simulink model "Tractor_HIT_Discrete"  (R2024a)
settings: Solver=ode1  StartTime=0.0  StopTime=60  FixedStep=0.001  RelTol=1e-3
values from neighbouring files (symbols this model uses):
  ANRtarget = 1.05    [Engine1204.sldd]    (also in Engine1204_init_r1.m; Engine2004.sldd; Engine2004_init.m; Engine3204.sldd)
  BackPrs = 3.0 4.2 5.5 7.0 8.5 10.0 11.5 12.5    [Engine1204.sldd]    (also in Engine1204_init_r1.m = [3.0, 4.2, 5.5, 7.0, 8.5, 10.0, 11.5, 12.5]; Engine2004.sldd = 3.0 4.2 5.5 7.0 8.5 10.0 11.5 12.5 13.5 14.5 15.0 15.5 16.0 ; Engine2004_init.m = [3.0,4.2,5.5,7.0,8.5,10.0,11.5,12.5,13.5,14.5,15.0,15.5,16.0; Engine3204.sldd = 3.0 4.5 6.0 7.5 9.0 10.5 12.0 13.0 13.8 14.4 14.8 15.2 15.6 )
  BackPrs_x = 50.0 100.0 150.0 200.0 250.0 300.0 350.0 400.0    [Engine1204.sldd]    (also in Engine1204_init_r1.m = [50:50:400]; Engine2004.sldd = 50.0 100.0 150.0 200.0 250.0 300.0 350.0 400.0 450.0 500.0 5; Engine2004_init.m = [50:50:800]; Engine3204.sldd = 100.0 200.0 300.0 400.0 500.0 600.0 700.0 800.0 900.0 1000.0)
  Bf = 0.38    [Engine1204.sldd]    (also in Engine2004.sldd; Engine3204.sldd)
  Br = 0.47    [Engine1204.sldd]    (also in Engine2004.sldd; Engine3204.sldd)
  BSFC = 320.0 285.0 275.0 280.0 290.0 300.0 310.0 260.0 225.0 215.0 220.0 228.0 240.0 250.0 235.0 208.0 202.0 205.0 212.0 222.0 232.0 230.0 205.0 200.0 204.0 210.0 220.0 230.0 232.0 207.0 203.0 206.0 213.0 224.0 235.0    [Engine1204.sldd]    (also in Engine1204_init_r1.m = [320,285,275,280,290,300,310; Engine2004.sldd = 315.0 280.0 270.0 275.0 285.0 295.0 305.0 255.0 220.0 210.0 ; Engine2004_init.m = [315,280,270,275,285,295,305; Engine3204.sldd = 310.0 275.0 265.0 270.0 280.0 290.0 300.0 250.0 215.0 205.0 )
  BSFC_x = 700.0 1200.0 1400.0 1600.0 1800.0 2000.0 2200.0    [Engine1204.sldd]    (also in Engine1204_init_r1.m = [700,1200,1400,1600,1800,2000,2200]; Engine2004.sldd = 800.0 1200.0 1400.0 1600.0 1800.0 2000.0 2200.0; Engine2004_init.m = [800,1200,1400,1600,1800,2000,2200]; Engine3204.sldd = 800.0 1000.0 1200.0 1400.0 1600.0 1800.0 2100.0)
  BSFC_y = 12.0 24.0 36.0 48.0 54.0    [Engine1204.sldd]    (also in Engine1204_init_r1.m = [12,24,36,48,54]; Engine2004.sldd = 20.0 40.0 60.0 80.0 100.0; Engine2004_init.m = [20,40,60,80,100]; Engine3204.sldd = 30.0 60.0 90.0 120.0 150.0)
  CO = 2.4 1.7 1.5 1.6 1.8 2.1 2.7 1.1 0.72 0.65 0.68 0.78 0.92 1.3 0.7 0.55 0.5 0.53 0.6 0.72 0.95 1.2 0.9 0.85 0.88 0.96 1.1 1.45 3.2 2.3 2.1 2.25 2.5 2.85 3.8    [Engine1204.sldd]    (also in Engine1204_init_r1.m = [; Engine2004.sldd = 2.3 1.63 1.44 1.54 1.73 2.02 2.56 1.05 0.68 0.61 0.64 0.74 0; Engine2004_init.m = [; Engine3204.sldd = 2.2 1.56 1.38 1.48 1.66 1.94 2.46 1.0 0.65 0.58 0.61 0.7 0.8)
  CO_x = 700.0 1200.0 1400.0 1600.0 1800.0 2000.0 2200.0    [Engine1204.sldd]    (also in Engine1204_init_r1.m = [700,1200,1400,1600,1800,2000,2200]; Engine2004.sldd = 800.0 1200.0 1400.0 1600.0 1800.0 2000.0 2200.0; Engine2004_init.m = [800,1200,1400,1600,1800,2000,2200]; Engine3204.sldd = 800.0 1000.0 1200.0 1400.0 1600.0 1800.0 2100.0)
  CO_y = 12.0 24.0 36.0 48.0 54.0    [Engine1204.sldd]    (also in Engine1204_init_r1.m = [12,24,36,48,54]; Engine2004.sldd = 20.0 40.0 60.0 80.0 100.0; Engine2004_init.m = [20,40,60,80,100]; Engine3204.sldd = 30.0 60.0 90.0 120.0 150.0)
  Df = 1.4    [Engine1204.sldd]    (also in Engine2004.sldd; Engine3204.sldd)
  dfmax = 0.1    [Engine1204.sldd]    (also in Engine2004.sldd; Engine3204.sldd)
  dfmin = 0.035    [Engine1204.sldd]    (also in Engine2004.sldd; Engine3204.sldd)
  DOCdPrs = 0.2 0.5 0.8 1.1 1.2    [Engine1204.sldd]    (also in Engine1204_init_r1.m = [0.2  0.5  0.8  1.1  1.2]; Engine2004.sldd = 0.25 0.55 0.85 1.15 1.3; Engine2004_init.m = [0.25,0.55,0.85,1.15,1.30]; Engine3204.sldd = 0.25 0.55 0.85 1.15 1.3 1.45)
  DOCdPrs_x = 50.0 150.0 250.0 350.0 400.0    [Engine1204.sldd]    (also in Engine1204_init_r1.m = [50  150  250  350  400]; Engine2004.sldd = 100.0 250.0 400.0 600.0 800.0; Engine2004_init.m = [100 250 400 600 800]; Engine3204.sldd = 100.0 250.0 400.0 600.0 800.0 1200.0)
  DPFdPrs = 0.3 0.5 0.7 0.9 0.6 1.0 1.4 1.8 0.9 1.5 2.1 2.6 1.2 2.0 2.7 2.8    [Engine1204.sldd]    (also in Engine1204_init_r1.m = [0.3  0.5  0.7  0.9; Engine2004.sldd = 0.35 0.6 0.85 1.1 0.7 1.15 1.6 2.0 1.05 1.7 2.3 2.5 1.4 2.2 ; Engine2004_init.m = [0.35,0.60,0.85,1.10; Engine3204.sldd = 0.35 0.7 1.05 1.4 1.7 2.0 2.2 2.4 2.55 2.65 2.7 2.75 0.6 1.1)
  DPFdPrs_x = 100.0 200.0 300.0 400.0    [Engine1204.sldd]    (also in Engine1204_init_r1.m = [100: 100 : 400]; Engine2004.sldd = 100.0 300.0 500.0 700.0; Engine2004_init.m = [100:200:700]; Engine3204.sldd = 100.0 200.0 300.0 400.0 500.0 600.0 700.0 800.0 900.0 1000.0)
  DPFdPrs_y = 0.0 6.0 12.0 20.0    [Engine1204.sldd]    (also in Engine1204_init_r1.m = [0 6 12 20 ]; Engine2004.sldd = 0.0 8.0 16.0 24.0; Engine2004_init.m = [0 8 16 24]; Engine3204.sldd = 0.0 10.0 20.0 30.0)
  DPFSootBurn = 0.0 0.0 0.0 0.0 0.0 0.2 0.4 0.6 0.8 1.0 1.2 2.4 3.6 4.8 6.0 6.0 12.0 18.0 24.0 30.0 12.0 24.0 36.0 48.0 60.0 20.0 40.0 60.0 80.0 100.0 22.0 44.0 66.0 88.0 110.0    [Engine1204.sldd]    (also in Engine1204_init_r1.m = [0,0,0,0,0; Engine2004.sldd = 0.0 0.0 0.0 0.0 0.0 0.5 1.0 1.5 2.0 2.5 3.0 6.0 9.0 12.0 15.; Engine2004_init.m = [0,0,0,0,0; Engine3204.sldd = 0.0 0.0 0.0 0.0 0.0 0.5 1.0 1.5 2.0 2.5 3.0 6.0 9.0 12.0 15.)
  DPFSootBurn_x = 100.0 200.0 300.0 400.0 500.0    [Engine1204.sldd]    (also in Engine1204_init_r1.m = [100,200,300,400,500]; Engine2004.sldd = 200.0 300.0 400.0 500.0 650.0; Engine2004_init.m = [200,300,400,500,650]; Engine3204.sldd = 200.0 300.0 400.0 500.0 650.0)
  DPFSootBurn_y = 400.0 450.0 500.0 550.0 600.0 650.0 680.0    [Engine1204.sldd]    (also in Engine1204_init_r1.m = [400,450,500,550,600,650,680]; Engine2004.sldd; Engine2004_init.m = [400,450,500,550,600,650,680]; Engine3204.sldd)
  Dr = 1.8    [Engine1204.sldd]    (also in Engine2004.sldd; Engine3204.sldd)
  drmax = 0.12    [Engine1204.sldd]    (also in Engine2004.sldd; Engine3204.sldd)
  drmin = 0.04    [Engine1204.sldd]    (also in Engine2004.sldd; Engine3204.sldd)
  EGRKi = 0.03    [Engine1204.sldd]    (also in Engine1204_init_r1.m; Engine2004.sldd; Engine2004_init.m; Engine3204.sldd)
  EGRKp = 3.5999999999999996    [Engine1204.sldd]    (also in Engine1204_init_r1.m = 3.6; Engine2004.sldd; Engine2004_init.m = 3.6; Engine3204.sldd)
  EGRMax = 1.0    [Engine1204.sldd]    (also in Engine1204_init_r1.m = 1; Engine2004.sldd; Engine2004_init.m = 1; Engine3204.sldd)
  EGRMin = 0.0    [Engine1204.sldd]    (also in Engine1204_init_r1.m = 0; Engine2004.sldd; Engine2004_init.m = 0; Engine3204.sldd)
  EGRRatio = 0.0 0.0 0.0 0.0 0.0 0.0 0.0 0.0 0.04 0.03 0.03 0.02 0.02 0.01 0.0 0.08 0.07 0.06 0.05 0.04 0.03 0.0 0.13 0.12 0.11 0.1 0.09 0.08 0.0 0.18 0.17 0.16 0.15 0.14 0.13 0.0 0.22 0.21 0.2 0.19 0.18 0.17    [Engine1204.sldd]    (also in Engine1204_init_r1.m = [; Engine2004.sldd; Engine2004_init.m = [; Engine3204.sldd)
  EGRRatio_x = 700.0 1200.0 1400.0 1600.0 1800.0 2000.0 2200.0    [Engine1204.sldd]    (also in Engine1204_init_r1.m = [700,1200,1400,1600,1800,2000,2200]; Engine2004.sldd = 800.0 1200.0 1400.0 1600.0 1800.0 2000.0 2200.0; Engine2004_init.m = [800,1200,1400,1600,1800,2000,2200]; Engine3204.sldd = 800.0 1000.0 1200.0 1400.0 1600.0 1800.0 2100.0)
  EGRRatio_y = 0.0 20.0 40.0 60.0 80.0 100.0    [Engine1204.sldd]    (also in Engine1204_init_r1.m = [0,20,40,60,80,100]; Engine2004.sldd; Engine2004_init.m = [0,20,40,60,80,100]; Engine3204.sldd)
  EGRTgt = 0.25 0.22 0.2 0.18 0.16 0.12 0.1 0.2 0.18 0.15 0.14 0.12 0.1 0.08 0.12 0.13 0.1 0.09 0.08 0.06 0.04 0.08 0.09 0.07 0.06 0.05 0.03 0.02 0.05 0.06 0.04 0.03 0.02 0.01 0.0    [Engine1204.sldd]    (also in Engine1204_init_r1.m = [0.25,0.22,0.20,0.18,0.16,0.12,0.10; Engine2004.sldd = 0.24 0.21 0.19 0.17 0.15 0.11 0.09 0.19 0.17 0.14 0.13 0.11 ; Engine2004_init.m = [0.24,0.21,0.19,0.17,0.15,0.11,0.09; Engine3204.sldd = 0.23 0.2 0.18 0.16 0.14 0.1 0.08 0.18 0.16 0.13 0.12 0.1 0.0)
  EGRTgt_x = 700.0 1200.0 1400.0 1600.0 1800.0 2000.0 2200.0    [Engine1204.sldd]    (also in Engine1204_init_r1.m = [700,1200,1400,1600,1800,2000,2200]; Engine2004.sldd = 800.0 1200.0 1400.0 1600.0 1800.0 2000.0 2200.0; Engine2004_init.m = [800,1200,1400,1600,1800,2000,2200]; Engine3204.sldd = 800.0 1000.0 1200.0 1400.0 1600.0 1800.0 2100.0)
  EGRTgt_y = 12.0 24.0 36.0 48.0 54.0    [Engine1204.sldd]    (also in Engine1204_init_r1.m = [12,24,36,48,54]; Engine2004.sldd = 20.0 40.0 60.0 80.0 100.0; Engine2004_init.m = [20,40,60,80,100]; Engine3204.sldd = 30.0 60.0 90.0 120.0 150.0)
  EGT = 197.0 257.0 287.0 297.0 287.0 267.0 247.0 267.0 357.0 397.0 407.0 392.0 367.0 347.0 337.0 437.0 472.0 482.0 462.0 437.0 407.0 367.0 477.0 502.0 512.0 492.0 467.0 437.0 377.0 487.0 510.0 520.0 500.0 477.0 447.0    [Engine1204.sldd]    (also in Engine1204_init_r1.m = [470,530,560,570,560,540,520; Engine2004.sldd = 187.0 247.0 277.0 287.0 277.0 257.0 237.0 257.0 347.0 387.0 ; Engine2004_init.m = [460,520,550,560,550,530,510; Engine3204.sldd = 307.0 327.0 338.0 327.0 307.0 277.0 237.0 322.0 337.0 332.0 )
  EGT_x = 700.0 1200.0 1400.0 1600.0 1800.0 2000.0 2200.0    [Engine1204.sldd]    (also in Engine1204_init_r1.m = [700,1200,1400,1600,1800,2000,2200]; Engine2004.sldd = 800.0 1200.0 1400.0 1600.0 1800.0 2000.0 2200.0; Engine2004_init.m = [800,1200,1400,1600,1800,2000,2200]; Engine3204.sldd = 800.0 1000.0 1200.0 1400.0 1600.0 1800.0 2100.0)
  EGT_y = 12.0 24.0 36.0 48.0 54.0    [Engine1204.sldd]    (also in Engine1204_init_r1.m = [12,24,36,48,54]; Engine2004.sldd = 20.0 40.0 60.0 80.0 100.0; Engine2004_init.m = [20,40,60,80,100]; Engine3204.sldd = 30.0 60.0 90.0 120.0 150.0)
  EngCsup = 0.35594 0.35501499999999997 0.353535 0.35242500000000004 0.351685 0.35150000000000003 0.35187 0.352795 0.35446 0.356865    [Engine1204.sldd]    (also in Engine2004.sldd; Engine3204.sldd)
  EngineSpdTgt = 700.0 850.0 1000.0 1150.0 1300.0 1450.0 1600.0 1750.0 1900.0 2050.0 2200.0    [Engine1204.sldd]    (also in Engine1204_init_r1.m = [700:150:2200]; Engine2004.sldd; Engine2004_init.m = [700:150:2200]; Engine3204.sldd = 800.0 930.0 1060.0 1190.0 1320.0 1450.0 1580.0 1710.0 1840.0)
  EngineSpdTgt_x = 0.0 10.0 20.0 30.0 40.0 50.0 60.0 70.0 80.0 90.0 100.0    [Engine1204.sldd]    (also in Engine1204_init_r1.m = [0:10:100]; Engine2004.sldd; Engine2004_init.m = [0:10:100]; Engine3204.sldd)
  EngineTrq = 70.0 110.0 130.0 125.0 115.0 100.0 85.0 180.0 280.0 320.0 310.0 285.0 250.0 220.0 260.0 370.0 410.0 395.0 365.0 320.0 280.0 300.0 420.0 450.0 435.0 400.0 350.0 300.0 310.0 435.0 460.0 445.0 410.0 355.0 305.0    [Engine1204.sldd]    (also in Engine1204_init_r1.m = [70,110,130,125,115,100,85; Engine2004.sldd = 130.0 200.0 240.0 230.0 210.0 180.0 150.0 320.0 480.0 550.0 ; Engine2004_init.m = [130,200,240,230,210,180,150; Engine3204.sldd = 210.0 320.0 380.0 360.0 330.0 290.0 240.0 510.0 760.0 870.0 )
  EngineTrq_x = 700.0 1200.0 1400.0 1600.0 1800.0 2000.0 2200.0    [Engine1204.sldd]    (also in Engine1204_init_r1.m = [700,1200,1400,1600,1800,2000,2200]; Engine2004.sldd = 800.0 1200.0 1400.0 1600.0 1800.0 2000.0 2200.0; Engine2004_init.m = [800,1200,1400,1600,1800,2000,2200]; Engine3204.sldd = 800.0 1000.0 1200.0 1400.0 1600.0 1800.0 2100.0)
  EngineTrq_y = 12.0 24.0 36.0 48.0 54.0    [Engine1204.sldd]    (also in Engine1204_init_r1.m = [12,24,36,48,54]; Engine2004.sldd = 20.0 40.0 60.0 80.0 100.0; Engine2004_init.m = [20,40,60,80,100]; Engine3204.sldd = 30.0 60.0 90.0 120.0 150.0)
  EngSpd = 800.0 1000.0 1200.0 1400.0 1600.0 1800.0 2000.0 2200.0 2400.0 2600.0    [Engine1204.sldd]    (also in Engine2004.sldd; Engine3204.sldd)
  EngTrq = 667.0 700.0 768.0 830.0 885.0 860.0 789.0 690.0 542.0 352.0    [Engine1204.sldd]    (also in Engine2004.sldd; Engine3204.sldd)
  etaCO = 0.0 0.0 0.0 0.0 0.6 0.45 0.3 0.15 0.92 0.85 0.75 0.6 0.98 0.95 0.9 0.82 0.99 0.97 0.94 0.88    [Engine1204.sldd]    (also in Engine1204_init_r1.m = [0.00	0.00	0.00	0.00; Engine2004.sldd; Engine2004_init.m = [0.00	0.00	0.00	0.00; Engine3204.sldd)
  etaCO_x = 10000.0 25000.0 40000.0 60000.0    [Engine1204.sldd]    (also in Engine1204_init_r1.m = [10000  25000  40000  60000]; Engine2004.sldd; Engine2004_init.m = [10000 25000 40000 60000]; Engine3204.sldd)
  etaCO_y = 120.0 200.0 280.0 360.0 450.0    [Engine1204.sldd]    (also in Engine1204_init_r1.m = [120, 200, 280, 360, 450]; Engine2004.sldd; Engine2004_init.m = [120,200,280,360,450]; Engine3204.sldd)
  etaHC = 0.0 0.0 0.0 0.0 0.5 0.35 0.2 0.1 0.88 0.8 0.68 0.5 0.96 0.92 0.86 0.75 0.98 0.95 0.91 0.83    [Engine1204.sldd]    (also in Engine1204_init_r1.m = [0.00	0.00	0.00	0.00; Engine2004.sldd; Engine2004_init.m = [0.00	0.00	0.00	0.00; Engine3204.sldd)
  etaHC_x = 10000.0 25000.0 40000.0 60000.0    [Engine1204.sldd]    (also in Engine1204_init_r1.m = [10000  25000  40000  60000]; Engine2004.sldd; Engine2004_init.m = [10000 25000 40000 60000]; Engine3204.sldd)
  etaHC_y = 120.0 200.0 280.0 360.0 450.0    [Engine1204.sldd]    (also in Engine1204_init_r1.m = [120, 200, 280, 360, 450]; Engine2004.sldd; Engine2004_init.m = [120,200,280,360,450]; Engine3204.sldd)
  etaNO2 = 0.0 0.0 0.0 0.0 0.2 0.15 0.1 0.05 0.4 0.33 0.25 0.18 0.55 0.48 0.4 0.3 0.6 0.53 0.45 0.35    [Engine1204.sldd]    (also in Engine1204_init_r1.m = [0.00	0.00	0.00	0.00; Engine2004.sldd; Engine2004_init.m = [0.00	0.00	0.00	0.00; Engine3204.sldd)
  etaNO2_x = 10000.0 25000.0 40000.0 60000.0    [Engine1204.sldd]    (also in Engine1204_init_r1.m = [10000  25000  40000  60000]; Engine2004.sldd; Engine2004_init.m = [10000 25000 40000 60000]; Engine3204.sldd)
  etaNO2_y = 120.0 200.0 280.0 360.0 450.0    [Engine1204.sldd]    (also in Engine1204_init_r1.m = [120, 200, 280, 360, 450]; Engine2004.sldd; Engine2004_init.m = [120,200,280,360,450]; Engine3204.sldd)
  etaPM = 0.995 0.992 0.988 0.98 0.996 0.994 0.99 0.985 0.997 0.995 0.992 0.988    [Engine1204.sldd]    (also in Engine1204_init_r1.m = [0.995  0.992  0.988  0.980; Engine2004.sldd; Engine2004_init.m = [0.995  0.992  0.988  0.980; Engine3204.sldd)
  etaPM_x = 10000.0 25000.0 40000.0 60000.0    [Engine1204.sldd]    (also in Engine1204_init_r1.m = [10000  25000  40000  60000]; Engine2004.sldd; Engine2004_init.m = [10000 25000 40000 60000]; Engine3204.sldd)
  etaPM_y = 150.0 300.0 450.0    [Engine1204.sldd]    (also in Engine1204_init_r1.m = [150, 300, 450]; Engine2004.sldd; Engine2004_init.m = [150,300,450]; Engine3204.sldd)
  FuelCyleMax = 40.0 45.0 50.0 52.0 54.0 50.0 60.0 65.0 66.0 68.0 52.0 64.0 66.0 67.0 68.0 50.0 62.0 64.0 65.0 66.0 48.0 58.0 60.0 61.0 62.0 42.0 50.0 52.0 53.0 54.0 38.0 44.0 46.0 47.0 48.0    [Engine1204.sldd]    (also in Engine1204_init_r1.m = [40,45,50,52,54; Engine2004.sldd = 65.0 75.0 82.0 88.0 92.0 75.0 88.0 94.0 98.0 102.0 78.0 92.0; Engine2004_init.m = [65,75,82,88,92; Engine3204.sldd = 95.0 110.0 125.0 140.0 155.0 110.0 130.0 145.0 160.0 175.0 1)
  FuelCyleMax_x = 80.0 140.0 200.0 260.0 320.0    [Engine1204.sldd]    (also in Engine1204_init_r1.m = [80,140,200,260,320]; Engine2004.sldd = 150.0 300.0 450.0 600.0 750.0; Engine2004_init.m = [150,300,450,600,750]; Engine3204.sldd = 250.0 500.0 750.0 1000.0 1300.0)
  FuelCyleMax_y = 700.0 1200.0 1400.0 1600.0 1800.0 2000.0 2200.0    [Engine1204.sldd]    (also in Engine1204_init_r1.m = [700,1200,1400,1600,1800,2000,2200]; Engine2004.sldd = 800.0 1200.0 1400.0 1600.0 1800.0 2000.0 2200.0; Engine2004_init.m = [800,1200,1400,1600,1800,2000,2200]; Engine3204.sldd = 800.0 1000.0 1200.0 1400.0 1600.0 1800.0 2100.0)
  FuelCyleMaxSw = 0.0    [Engine1204.sldd]    (also in Engine1204_init_r1.m = 0; Engine2004.sldd; Engine2004_init.m = 0; Engine3204.sldd)
  FuelCyleMin = 10.0    [Engine1204.sldd]    (also in Engine1204_init_r1.m = 10; Engine2004.sldd = 12.0; Engine2004_init.m = 12; Engine3204.sldd = 15.0)
  FuelKd = 0.0    [Engine1204.sldd]    (also in Engine1204_init_r1.m = 0; Engine2004.sldd; Engine2004_init.m = 0; Engine3204.sldd)
  FuelKi = 0.0162    [Engine1204.sldd]    (also in Engine1204_init_r1.m; Engine2004.sldd = 0.0198; Engine2004_init.m = 0.0198; Engine3204.sldd = 0.025199999999999997)
  FuelKp = 0.054    [Engine1204.sldd]    (also in Engine1204_init_r1.m; Engine2004.sldd = 0.066; Engine2004_init.m = 0.066; Engine3204.sldd = 0.083999999999999991)
  g = 9.81    [Engine1204.sldd]    (also in Engine2004.sldd; Engine3204.sldd)
  GearA = -2.9 0.0 6.0 2.5 1.0    [Engine1204.sldd]    (also in Engine2004.sldd; Engine3204.sldd)
  GearAC = -1.0 0.0 1.0 2.0 3.0    [Engine1204.sldd]    (also in Engine2004.sldd; Engine3204.sldd)
  GearFront = 17.574    [Engine1204.sldd]    (also in Engine2004.sldd; Engine3204.sldd)
  GearM = 2.33 1.75 1.4 1.0    [Engine1204.sldd]    (also in Engine2004.sldd; Engine3204.sldd)
  GearMC = 1.0 2.0 3.0 4.0    [Engine1204.sldd]    (also in Engine2004.sldd; Engine3204.sldd)
  GearRef = 14.6    [Engine1204.sldd]    (also in Engine2004.sldd; Engine3204.sldd)
  HC = 0.85 0.6 0.52 0.55 0.62 0.7 0.9 0.4 0.22 0.2 0.21 0.26 0.32 0.48 0.25 0.18 0.17 0.18 0.21 0.26 0.36 0.32 0.24 0.23 0.25 0.28 0.33 0.42 0.55 0.42 0.4 0.43 0.48 0.54 0.68    [Engine1204.sldd]    (also in Engine1204_init_r1.m = [; Engine2004.sldd = 0.82 0.58 0.5 0.53 0.6 0.68 0.87 0.38 0.21 0.19 0.2 0.24 0.3; Engine2004_init.m = [; Engine3204.sldd = 0.8 0.56 0.48 0.51 0.58 0.66 0.84 0.37 0.2 0.18 0.19 0.23 0.)
  HC_x = 700.0 1200.0 1400.0 1600.0 1800.0 2000.0 2200.0    [Engine1204.sldd]    (also in Engine1204_init_r1.m = [700,1200,1400,1600,1800,2000,2200]; Engine2004.sldd = 800.0 1200.0 1400.0 1600.0 1800.0 2000.0 2200.0; Engine2004_init.m = [800,1200,1400,1600,1800,2000,2200]; Engine3204.sldd = 800.0 1000.0 1200.0 1400.0 1600.0 1800.0 2100.0)
  HC_y = 12.0 24.0 36.0 48.0 54.0    [Engine1204.sldd]    (also in Engine1204_init_r1.m = [12,24,36,48,54]; Engine2004.sldd = 20.0 40.0 60.0 80.0 100.0; Engine2004_init.m = [20,40,60,80,100]; Engine3204.sldd = 30.0 60.0 90.0 120.0 150.0)
  hf = 0.35    [Engine1204.sldd]    (also in Engine2004.sldd; Engine3204.sldd)
  hr = 0.4    [Engine1204.sldd]    (also in Engine2004.sldd; Engine3204.sldd)
  IdleEngSpd = 700.0    [Engine1204.sldd]    (also in Engine2004.sldd; Engine3204.sldd)
  IdleThrottle = 0.3    [Engine1204.sldd]    (also in Engine2004.sldd; Engine3204.sldd)
  Inertia = 0.9    [Engine1204.sldd]    (also in Engine1204_init_r1.m; Engine2004.sldd = 1.4; Engine2004_init.m = 1.4; Engine3204.sldd = 2.0)
  Intake = 80.0 140.0 160.0 180.0 190.0 195.0 200.0 130.0 210.0 240.0 260.0 270.0 275.0 280.0 170.0 270.0 310.0 330.0 340.0 345.0 350.0 190.0 320.0 360.0 380.0 390.0 395.0 400.0 200.0 340.0 380.0 400.0 410.0 415.0 420.0    [Engine1204.sldd]    (also in Engine1204_init_r1.m = [80,140,160,180,190,195,200; Engine2004.sldd = 160.0 240.0 280.0 310.0 330.0 340.0 350.0 250.0 380.0 440.0 ; Engine2004_init.m = [160,240,280,310,330,340,350; Engine3204.sldd = 280.0 420.0 490.0 540.0 570.0 585.0 600.0 430.0 660.0 760.0 )
  Intake_x = 700.0 1200.0 1400.0 1600.0 1800.0 2000.0 2200.0    [Engine1204.sldd]    (also in Engine1204_init_r1.m = [700,1200,1400,1600,1800,2000,2200]; Engine2004.sldd = 800.0 1200.0 1400.0 1600.0 1800.0 2000.0 2200.0; Engine2004_init.m = [800,1200,1400,1600,1800,2000,2200]; Engine3204.sldd = 800.0 1000.0 1200.0 1400.0 1600.0 1800.0 2100.0)
  Intake_y = 12.0 24.0 36.0 48.0 54.0    [Engine1204.sldd]    (also in Engine1204_init_r1.m = [12,24,36,48,54]; Engine2004.sldd = 20.0 40.0 60.0 80.0 100.0; Engine2004_init.m = [20,40,60,80,100]; Engine3204.sldd = 30.0 60.0 90.0 120.0 150.0)
  IntakePrs = 1.0 1.1 1.22 1.35 1.48 1.6 1.7 1.0 1.12 1.24 1.37 1.5 1.62 1.72 1.0 1.13 1.25 1.38 1.51 1.63 1.73 1.0 1.14 1.26 1.39 1.52 1.64 1.74 1.0 1.15 1.27 1.4 1.53 1.65 1.75 1.0 1.16 1.28 1.41 1.54 1.66 1.76    [Engine1204.sldd]    (also in Engine1204_init_r1.m = [; Engine2004.sldd = 1.0 1.11 1.23 1.36 1.49 1.61 1.71 1.0 1.13 1.25 1.38 1.51 1.; Engine2004_init.m = [; Engine3204.sldd = 1.0 1.12 1.24 1.37 1.5 1.62 1.72 1.0 1.14 1.26 1.39 1.52 1.6)
  IntakePrs_x = 700.0 1200.0 1400.0 1600.0 1800.0 2000.0 2200.0    [Engine1204.sldd]    (also in Engine1204_init_r1.m = [700,1200,1400,1600,1800,2000,2200]; Engine2004.sldd = 800.0 1200.0 1400.0 1600.0 1800.0 2000.0 2200.0; Engine2004_init.m = [800,1200,1400,1600,1800,2000,2200]; Engine3204.sldd = 800.0 1000.0 1200.0 1400.0 1600.0 1800.0 2100.0)
  IntakePrs_y = 0.0 20.0 40.0 60.0 80.0 100.0    [Engine1204.sldd]    (also in Engine1204_init_r1.m = [0,20,40,60,80,100]; Engine2004.sldd; Engine2004_init.m = [0,20,40,60,80,100]; Engine3204.sldd)
  IntakePrsInit = 1.35    [Engine1204.sldd]    (also in Engine1204_init_r1.m; Engine2004.sldd; Engine2004_init.m; Engine3204.sldd)
  IntakeSw = 0    [Engine1204.sldd]    (also in Engine1204_init_r1.m = false; Engine2004.sldd; Engine2004_init.m = false; Engine3204.sldd)
  IntakeTC = 0.1    [Engine1204.sldd]    (also in Engine1204_init_r1.m; Engine2004.sldd; Engine2004_init.m; Engine3204.sldd)
  IntakeTemp = 25.0 28.0 30.0 32.0 34.0 36.0 38.0 25.0 38.0 40.0 42.0 44.0 46.0 48.0 25.0 48.0 50.0 52.0 54.0 56.0 58.0 25.0 58.0 60.0 62.0 64.0 66.0 68.0 25.0 66.0 68.0 70.0 72.0 74.0 76.0 25.0 72.0 74.0 76.0 78.0 80.0 82.0    [Engine1204.sldd]    (also in Engine1204_init_r1.m = [; Engine2004.sldd = 25.0 29.0 31.0 33.0 35.0 37.0 39.0 25.0 39.0 41.0 43.0 45.0 ; Engine2004_init.m = [; Engine3204.sldd = 25.0 30.0 32.0 34.0 36.0 38.0 40.0 25.0 40.0 42.0 44.0 46.0 )
  IntakeTemp_x = 700.0 1200.0 1400.0 1600.0 1800.0 2000.0 2200.0    [Engine1204.sldd]    (also in Engine1204_init_r1.m = [700,1200,1400,1600,1800,2000,2200]; Engine2004.sldd = 800.0 1200.0 1400.0 1600.0 1800.0 2000.0 2200.0; Engine2004_init.m = [800,1200,1400,1600,1800,2000,2200]; Engine3204.sldd = 800.0 1000.0 1200.0 1400.0 1600.0 1800.0 2100.0)
  IntakeTemp_y = 0.0 20.0 40.0 60.0 80.0 100.0    [Engine1204.sldd]    (also in Engine1204_init_r1.m = [0,20,40,60,80,100]; Engine2004.sldd; Engine2004_init.m = [0,20,40,60,80,100]; Engine3204.sldd)
  IntakeTempInit = 45.0    [Engine1204.sldd]    (also in Engine1204_init_r1.m = 45; Engine2004.sldd; Engine2004_init.m = 45; Engine3204.sldd)
  Jf = 180.0    [Engine1204.sldd]    (also in Engine2004.sldd; Engine3204.sldd)
  Jr = 450.0    [Engine1204.sldd]    (also in Engine2004.sldd; Engine3204.sldd)
  L = 2.75    [Engine1204.sldd]    (also in Engine2004.sldd; Engine3204.sldd)
  LiftTorque = 5000.0    [Engine1204.sldd]    (also in Engine2004.sldd; Engine3204.sldd)
  LoadTrqManu = 200.0    [Engine1204.sldd]    (also in Engine1204_init_r1.m = 200; Engine2004.sldd = 400.0; Engine2004_init.m = 400; Engine3204.sldd = 800.0)
  LoadTrqSW = 1    [Engine1204.sldd]    (also in Engine1204_init_r1.m = true; Engine2004.sldd; Engine2004_init.m = true; Engine3204.sldd = 0)
  M_I = 2500.0    [Engine1204.sldd]    (also in Engine2004.sldd; Engine3204.sldd)
  M_T = 6500.0    [Engine1204.sldd]    (also in Engine2004.sldd; Engine3204.sldd)
  MaxEngSpd = 2600.0    [Engine1204.sldd]    (also in Engine2004.sldd; Engine3204.sldd)
  NH3StoreMax = 0.0 1.2 2.0 2.4 2.2 1.7 1.1    [Engine1204.sldd]    (also in Engine1204_init_r1.m = [0  1.2  2.0  2.4  2.2  1.7  1.1]; Engine2004.sldd = 0.0 1.7 2.9 3.5 3.2 2.5 1.6; Engine2004_init.m = [0, 1.7, 2.9, 3.5, 3.2, 2.5, 1.6]; Engine3204.sldd = 0.0 2.2 3.8 4.5 4.2 3.3 2.1)
  NH3StoreMax_x = 180.0 220.0 260.0 300.0 340.0 380.0 420.0    [Engine1204.sldd]    (also in Engine1204_init_r1.m = [180  220  260  300  340  380  420]; Engine2004.sldd; Engine2004_init.m = [180 220 260 300 340 380 420]; Engine3204.sldd)
  NOx = 6.2 7.0 7.4 7.2 6.8 6.4 6.0 7.5 8.4 8.8 8.6 8.2 7.7 7.2 8.2 9.1 9.5 9.3 8.9 8.4 7.9 7.6 8.5 8.8 8.6 8.2 7.7 7.2 7.0 7.8 8.1 7.9 7.5 7.0 6.5    [Engine1204.sldd]    (also in Engine1204_init_r1.m = [6.2,7.0,7.4,7.2,6.8,6.4,6.0; Engine2004.sldd = 6.1 6.9 7.3 7.1 6.7 6.3 5.9 7.4 8.3 8.7 8.5 8.1 7.6 7.1 8.1 ; Engine2004_init.m = [6.1,6.9,7.3,7.1,6.7,6.3,5.9; Engine3204.sldd = 5.9 6.7 7.1 6.9 6.5 6.1 5.7 7.2 8.1 8.5 8.3 7.9 7.4 6.9 7.9 )
  NOx_x = 700.0 1200.0 1400.0 1600.0 1800.0 2000.0 2200.0    [Engine1204.sldd]    (also in Engine1204_init_r1.m = [700,1200,1400,1600,1800,2000,2200]; Engine2004.sldd = 800.0 1200.0 1400.0 1600.0 1800.0 2000.0 2200.0; Engine2004_init.m = [800,1200,1400,1600,1800,2000,2200]; Engine3204.sldd = 800.0 1000.0 1200.0 1400.0 1600.0 1800.0 2100.0)
  NOx_y = 12.0 24.0 36.0 48.0 54.0    [Engine1204.sldd]    (also in Engine1204_init_r1.m = [12,24,36,48,54]; Engine2004.sldd = 20.0 40.0 60.0 80.0 100.0; Engine2004_init.m = [20,40,60,80,100]; Engine3204.sldd = 30.0 60.0 90.0 120.0 150.0)
  NOxFac = 1.0 0.88 0.76 0.64 0.54 0.46 0.4    [Engine1204.sldd]    (also in Engine1204_init_r1.m = [1.00, 0.88, 0.76, 0.64, 0.54, 0.46, 0.40]; Engine2004.sldd; Engine2004_init.m = [1.00,0.88,0.76,0.64,0.54,0.46,0.40]; Engine3204.sldd)
  NOxFac_x = 0.0 0.05 0.1 0.15 0.19999999999999998 0.25 0.3    [Engine1204.sldd]    (also in Engine1204_init_r1.m = [0: 0.05 : 0.3]; Engine2004.sldd; Engine2004_init.m = [0:0.05:0.3]; Engine3204.sldd)
  NumCyl = 6.0    [Engine1204.sldd]    (also in Engine1204_init_r1.m = 6; Engine2004.sldd; Engine2004_init.m = 6; Engine3204.sldd)
  O2 = 16.5 16.0 15.8 15.5 15.2 14.8 14.5 13.0 12.2 11.8 11.5 11.2 10.8 10.5 9.5 8.6 8.0 7.7 7.4 7.0 6.7 7.0 6.2 5.6 5.3 5.0 4.7 4.4 6.0 5.3 4.8 4.5 4.2 4.0 3.8    [Engine1204.sldd]    (also in Engine1204_init_r1.m = [16.5,16.0,15.8,15.5,15.2,14.8,14.5; Engine2004.sldd = 16.3 15.8 15.6 15.3 15.0 14.6 14.3 12.8 12.0 11.6 11.3 11.0 ; Engine2004_init.m = [16.3,15.8,15.6,15.3,15.0,14.6,14.3; Engine3204.sldd = 16.0 15.5 15.3 15.0 14.7 14.3 14.0 12.5 11.7 11.3 11.0 10.7 )
  O2_x = 700.0 1200.0 1400.0 1600.0 1800.0 2000.0 2200.0    [Engine1204.sldd]    (also in Engine1204_init_r1.m = [700,1200,1400,1600,1800,2000,2200]; Engine2004.sldd = 800.0 1200.0 1400.0 1600.0 1800.0 2000.0 2200.0; Engine2004_init.m = [800,1200,1400,1600,1800,2000,2200]; Engine3204.sldd = 800.0 1000.0 1200.0 1400.0 1600.0 1800.0 2100.0)
  O2_y = 12.0 24.0 36.0 48.0 54.0    [Engine1204.sldd]    (also in Engine1204_init_r1.m = [12,24,36,48,54]; Engine2004.sldd = 20.0 40.0 60.0 80.0 100.0; Engine2004_init.m = [20,40,60,80,100]; Engine3204.sldd = 30.0 60.0 90.0 120.0 150.0)
  PM = 0.12 0.1 0.09 0.09 0.1 0.11 0.12 0.22 0.18 0.16 0.17 0.19 0.21 0.24 0.38 0.3 0.26 0.27 0.31 0.35 0.39 0.55 0.44 0.38 0.4 0.45 0.5 0.56 0.65 0.52 0.46 0.48 0.53 0.58 0.66    [Engine1204.sldd]    (also in Engine1204_init_r1.m = [0.12,0.10,0.09,0.09,0.10,0.11,0.12; Engine2004.sldd = 0.11 0.09 0.08 0.08 0.09 0.1 0.11 0.21 0.17 0.15 0.16 0.18 0; Engine2004_init.m = [0.11,0.09,0.08,0.08,0.09,0.10,0.11; Engine3204.sldd = 0.1 0.08 0.07 0.07 0.08 0.09 0.1 0.2 0.16 0.14 0.15 0.17 0.1)
  PM_x = 700.0 1200.0 1400.0 1600.0 1800.0 2000.0 2200.0    [Engine1204.sldd]    (also in Engine1204_init_r1.m = [700,1200,1400,1600,1800,2000,2200]; Engine2004.sldd = 800.0 1200.0 1400.0 1600.0 1800.0 2000.0 2200.0; Engine2004_init.m = [800,1200,1400,1600,1800,2000,2200]; Engine3204.sldd = 800.0 1000.0 1200.0 1400.0 1600.0 1800.0 2100.0)
  PM_y = 12.0 24.0 36.0 48.0 54.0    [Engine1204.sldd]    (also in Engine1204_init_r1.m = [12,24,36,48,54]; Engine2004.sldd = 20.0 40.0 60.0 80.0 100.0; Engine2004_init.m = [20,40,60,80,100]; Engine3204.sldd = 30.0 60.0 90.0 120.0 150.0)
  radps2rpm = 9.55    [Engine1204.sldd]    (also in Engine1204_init_r1.m; Engine2004.sldd; Engine2004_init.m; Engine3204.sldd)
  RailFuel = 400.0 600.0 700.0 700.0 650.0 600.0 550.0 600.0 800.0 900.0 900.0 850.0 800.0 750.0 700.0 1000.0 1100.0 1150.0 1100.0 1000.0 950.0 750.0 1200.0 1350.0 1350.0 1300.0 1200.0 1150.0 750.0 1300.0 1400.0 1450.0 1400.0 1300.0 1200.0    [Engine1204.sldd]    (also in Engine1204_init_r1.m = [400,600,700,700,650,600,550; Engine2004.sldd = 420.0 620.0 720.0 720.0 680.0 630.0 580.0 630.0 830.0 930.0 ; Engine2004_init.m = [420,620,720,720,680,630,580; Engine3204.sldd = 440.0 640.0 740.0 740.0 700.0 650.0 600.0 650.0 850.0 950.0 )
  RailFuel_x = 700.0 1200.0 1400.0 1600.0 1800.0 2000.0 2200.0    [Engine1204.sldd]    (also in Engine1204_init_r1.m = [700,1200,1400,1600,1800,2000,2200]; Engine2004.sldd = 800.0 1200.0 1400.0 1600.0 1800.0 2000.0 2200.0; Engine2004_init.m = [800,1200,1400,1600,1800,2000,2200]; Engine3204.sldd = 800.0 1000.0 1200.0 1400.0 1600.0 1800.0 2100.0)
  ... (+23 more)
undefined symbols (not defined in the file or in its folder): df, DiscIntNeverNeededParam, dr, MAP_AIR, MAP_EFF, MAP_EoCO, MAP_EoCO2, MAP_EoHC, MAP_EoNOx, MAP_EoPM, MAP_FUEL, MAP_FUELCMD, MAP_POWER, MAP_SPD, MAP_TEMPERATURE, NH3_MAX, R
libraries: simulink x9, slpidlib x5
(part 7 of 10)

== system Tractor_HIT_Discrete/WorkloadModel/Tires and Ground/CI_Calc ==
  Soil[-] : Inport
  moisture[%] : Inport  Port=2
  density[g/cm3] : Inport  Port=3
  Scene[-] : Inport  Port=4
  1 : Subsystem  Commented=on  TreatAsAtomicUnit=on
  2 : Subsystem  TreatAsAtomicUnit=on
  If : If  IfExpression=u1 == 0  ElseIfExpressions=u1 == 1,u1 == 2  ShowElse=off
  If Action Subsystem : Subsystem  TreatAsAtomicUnit=on
  If Action Subsystem1 : Subsystem  TreatAsAtomicUnit=on
  Merge : Merge  Inputs=3
  CI[kPa] : Outport
  wires:
  Soil[-]/1 -> If/1
  moisture[%]/1 -> [moisture]
  density[g/cm3]/1 -> [density]
  [moisture] -> If Action Subsystem/1(moisture[%])
  [density] -> If Action Subsystem/2(density[g/cm3])
  Merge/1 -> CI[kPa]/1
  If/1 -> If Action Subsystem/Action
  If Action Subsystem/1(CI) -> Merge/1
  If Action Subsystem1/1(CI) -> Merge/2
  [moisture] -> If Action Subsystem1/1(moisture[%])
  [density] -> If Action Subsystem1/2(density[g/cm3])
  2/1(CI) -> Merge/3
  [moisture] -> 2/1(moisture[%])
  [density] -> 2/2(density[g/cm3])
  If/3 -> 2/Action
  If/2 -> If Action Subsystem1/Action
  Scene[-]/1 -> If Action Subsystem/3(Scene[-])

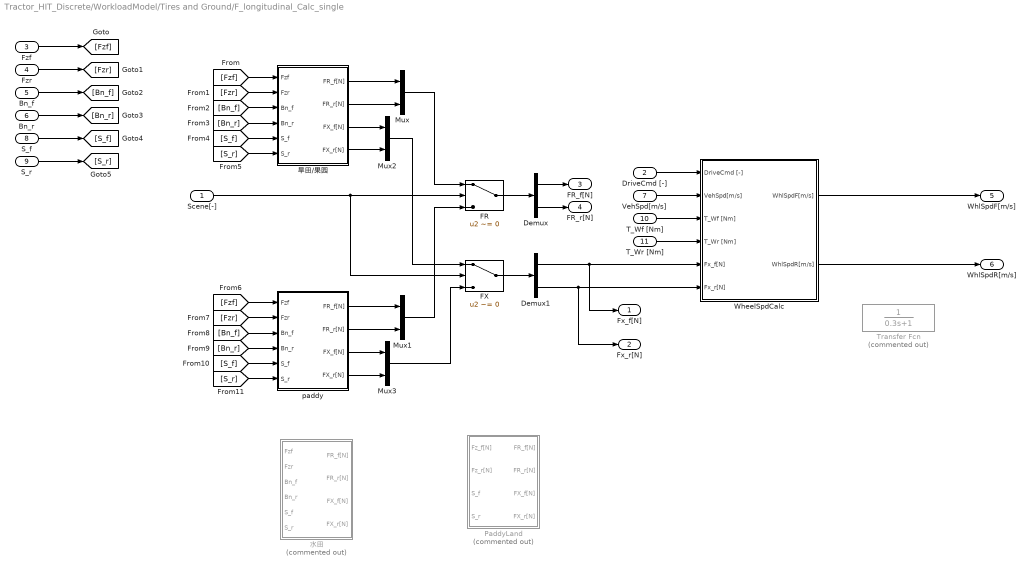
== system Tractor_HIT_Discrete/WorkloadModel/Tires and Ground/F_longitudinal_Calc_single ==
  Scene[-] : Inport
  DriveCmd [-] : Inport  Port=2
  Fzf : Inport  Port=3
  Fzr : Inport  Port=4
  Bn_f : Inport  Port=5
  Bn_r : Inport  Port=6
  VehSpd[m/s] : Inport  Port=7
  S_f : Inport  Port=8
  S_r : Inport  Port=9
  T_Wf [Nm] : Inport  Port=10
  T_Wr [Nm] : Inport  Port=11
  Demux : Demux  Outputs=2
  Demux1 : Demux  Outputs=2
  FR : Switch  Criteria=u2 ~= 0  SaturateOnIntegerOverflow=off  InputSameDT=off
  FX : Switch  Criteria=u2 ~= 0  SaturateOnIntegerOverflow=off  InputSameDT=off
  Mux{,1..3} (4 alike) : Mux  Inputs=2
  PaddyLand : Subsystem  Commented=on
  Transfer Fcn : TransferFcn  Commented=on  Denominator=[0.3 1]
  WheelSpdCalc : Subsystem
  paddy : Subsystem
  旱田/果园 : Subsystem
  水田 : Subsystem  Commented=on
  Fx_f[N] : Outport
  Fx_r[N] : Outport  Port=2
  FR_f[N] : Outport  Port=3
  FR_r[N] : Outport  Port=4
  WhlSpdF[m/s] : Outport  Port=5
  WhlSpdR[m/s] : Outport  Port=6
  wires:
  DriveCmd [-]/1 -> WheelSpdCalc/1(DriveCmd [-])
  T_Wf [Nm]/1 -> WheelSpdCalc/3(T_Wf [Nm])
  VehSpd[m/s]/1 -> WheelSpdCalc/2(VehSpd[m/s])
  T_Wr [Nm]/1 -> WheelSpdCalc/4(T_Wr [Nm])
  Scene[-]/1 -> FR/2, FX/2
  FR/1 -> Demux/1
  旱田/果园/1(FR_f[N]) -> Mux/1
  旱田/果园/2(FR_r[N]) -> Mux/2
  paddy/1(FR_f[N]) -> Mux1/1
  paddy/2(FR_r[N]) -> Mux1/2
  Mux1/1 -> FR/3
  Mux/1 -> FR/1
  Demux/1 -> FR_f[N]/1
  Demux/2 -> FR_r[N]/1
  FX/1 -> Demux1/1
  Demux1/1 -> Fx_f[N]/1, WheelSpdCalc/5(Fx_f[N])
  Demux1/2 -> Fx_r[N]/1, WheelSpdCalc/6(Fx_r[N])
  旱田/果园/3(FX_f[N]) -> Mux2/1
  旱田/果园/4(FX_r[N]) -> Mux2/2
  paddy/3(FX_f[N]) -> Mux3/1
  paddy/4(FX_r[N]) -> Mux3/2
  Mux3/1 -> FX/3
  Mux2/1 -> FX/1
  Fzf/1 -> [Fzf]
  Fzr/1 -> [Fzr]
  S_r/1 -> [S_r]
  S_f/1 -> [S_f]
  Bn_r/1 -> [Bn_r]
  Bn_f/1 -> [Bn_f]
  [Bn_r] -> 旱田/果园/4(Bn_r)
  [S_f] -> 旱田/果园/5(S_f)
  [S_r] -> 旱田/果园/6(S_r)
  [Bn_f] -> 旱田/果园/3(Bn_f)
  [Fzr] -> 旱田/果园/2(Fzr)
  [Fzf] -> 旱田/果园/1(Fzf)
  [Fzf] -> paddy/1(Fzf)
  [Fzr] -> paddy/2(Fzr)
  [Bn_f] -> paddy/3(Bn_f)
  [S_r] -> paddy/6(S_r)
  [S_f] -> paddy/5(S_f)
  [Bn_r] -> paddy/4(Bn_r)
  WheelSpdCalc/1(WhlSpdF[m/s]) -> WhlSpdF[m/s]/1
  WheelSpdCalc/2(WhlSpdR[m/s]) -> WhlSpdR[m/s]/1

== system Tractor_HIT_Discrete/WorkloadModel/Tires and Ground/Fz_Calc_single ==
  pitch_angle[rad] : Inport
  Add : Sum
  Add1 : Sum
  Constant : Constant  Value=M_T
  Constant1 : Constant  Value=g
  Constant2 : Constant  Value=L
  Constant3 : Constant  Value=L
  Constant4 : Constant  Value=Xof
  Constant5 : Constant  Value=Xor
  Constant6 : Constant  Value=Rr
  Constant7 : Constant  Value=Zor
  Cos : Trigonometry  Operator=cos
  Display : Display
  Display1 : Display
  Divide : Product  Inputs=*/
  Divide1 : Product  Inputs=*/
  Fz_Calc : Subsystem  Commented=on
  Gain : Gain  Gain=0.5
  Gain1 : Gain  Gain=0.5
  Product : Product
  Product2 : Product  Inputs=3
  Product3 : Product  Inputs=3
  Product4 : Product  Inputs=3
  Sin : Trigonometry
  Subtract : Sum  Inputs=+-
  Fzf : Outport
  Fzr : Outport  Port=2
  wires:
  pitch_angle[rad]/1 -> Sin/1, Cos/1
  Constant/1 -> Product/1
  Constant1/1 -> Product/2
  Constant2/1 -> Divide/2
  Constant3/1 -> Divide1/2
  Constant5/1 -> Product2/1
  Cos/1 -> Product2/2, Product3/2
  Product3/1 -> Subtract/1
  Product2/1 -> Add/1
  Constant4/1 -> Product3/3
  Add/1 -> Divide1/1
  Subtract/1 -> Divide/1
  Sin/1 -> Product4/3
  Product4/1 -> Add/2, Subtract/2
  Constant6/1 -> Add1/1
  Constant7/1 -> Add1/2
  Add1/1 -> Product4/2
  Divide1/1 -> Display1/1, Gain/1
  Divide/1 -> Display/1, Gain1/1
  Gain/1 -> Fzf/1
  Gain1/1 -> Fzr/1
  Product/1 -> Product4/1, Product3/1, Product2/3

== system Tractor_HIT_Discrete/WorkloadModel/Tires and Ground/Slip_calc ==
  VehSpd [m/s] : Inport
  WhlSpdF[m/s] : Inport  Port=2
  WhlSpdR[m/s] : Inport  Port=3
  Add : Sum
  Add1 : Sum
  Add2 : Sum  Inputs=+-
  Add3 : Sum  Inputs=+-
  Constant : Constant  Value=eps
  Divide : Product  Inputs=*/
  Divide1 : Product  Inputs=*/
  Max : MinMax  Function=max  Inputs=2
  Max1 : MinMax  Function=max  Inputs=2
  Scope : Scope  NumInputPorts=3
  SlipF [-] : Outport
  SlipR [-] : Outport  Port=2
  wires:
  Add3/1 -> Divide1/1
  Max/1 -> Add1/1
  Add2/1 -> Divide/1
  Constant/1 -> Add/2, Add1/2
  Max1/1 -> Add/1
  Add/1 -> Divide1/2
  Add1/1 -> Divide/2
  WhlSpdF[m/s]/1 -> Scope/2, Max/2, Add2/1
  VehSpd [m/s]/1 -> Scope/1, Max/1, Max1/1, Add3/2, Add2/2
  WhlSpdR[m/s]/1 -> Max1/2, Scope/3, Add3/1
  Divide1/1 -> SlipR [-]/1
  Divide/1 -> SlipF [-]/1

== system Tractor_HIT_Discrete/WorkloadModel/Tires and Ground/SlopeResistance_Calc ==
  note: SlopeResis_Calc
  Terrain[-] : Inport
  Constant2 : Constant  Value=M_T
  Fcn : Fcn  Expr=sin(u)
  Gain6 : Gain  Gain=pi/180
  Gain8 : Gain  Gain=g
  Multiport Switch : MultiPortSwitch  DataPortOrder=Zero-based contiguous  zeroidx=on  SaturateOnIntegerOverflow=off  InputSameDT=off
  Product2 : Product
  Sine Wave : Sin  Amplitude=5  Frequency=20  SampleTime=0
  Sine Wave1 : Sin  Amplitude=15  Frequency=10  SampleTime=0
  Sine Wave2 : Sin  Amplitude=30  Frequency=5  SampleTime=0
  SlopeResis[N] : Outport
  pitch_angle[rad] : Outport  Port=2
  wires:
  Sine Wave2/1 -> Multiport Switch/4
  Fcn/1 -> Product2/2
  Gain6/1 -> pitch_angle[rad]/1, Fcn/1
  Gain8/1 -> Product2/1
  Constant2/1 -> Gain8/1
  Multiport Switch/1 -> Gain6/1
  Sine Wave/1 -> Multiport Switch/2
  Sine Wave1/1 -> Multiport Switch/3
  Product2/1 -> SlopeResis[N]/1
  Terrain[-]/1 -> Multiport Switch/1

== system Tractor_HIT_Discrete/WorkloadModel/Transmission/EngSpdCalc ==
  Gear_R[-] : Inport
  DriveWhlSpd[m/s] : Inport  Port=2
  DriveWhlR[m] : Inport  Port=3
  Constant1 : Constant  Value=9.55
  Divide : Product  Inputs=*/
  Product : Product  Inputs=3
  Saturation1 : Saturate  UpperLimit=MaxEngSpd  LowerLimit=IdleEngSpd
  Scope2 : Scope  NumInputPorts=4
  EngSpd [rpm] : Outport
  wires:
  Product/1 -> Scope2/2, Divide/1
  Constant1/1 -> Product/3
  DriveWhlR[m]/1 -> Divide/2
  Divide/1 -> Scope2/3, Saturation1/1
  DriveWhlSpd[m/s]/1 -> Scope2/1, Product/2
  Gear_R[-]/1 -> Product/1
  Saturation1/1 -> Scope2/4, EngSpd [rpm]/1

== system Tractor_HIT_Discrete/WorkloadModel/Transmission/GearBox ==
  GearCmd[-] : Inport
  EngTrq [Nm] : Inport  Port=2
  1-D Lookup Table1 : Lookup_n-D  NumberOfTableDimensions=1  BreakpointsForDimension1=GearMC  Table=GearM  InternalRulePriority=Speed  RndMeth=Simplest
  1-D Lookup Table2 : Lookup_n-D  NumberOfTableDimensions=1  BreakpointsForDimension1=GearAC  Table=GearA  InternalRulePriority=Speed  RndMeth=Simplest
  1-D Lookup Table3 : Lookup_n-D  NumberOfTableDimensions=1  BreakpointsForDimension1=SlowFastC  Table=SlowFastGear  InternalRulePriority=Speed  RndMeth=Simplest
  Bus Selector : BusSelector  OutputSignals=FastSlowCmd,GearMCmd,GearACmd
  Effi : Constant  Value=TransEff
  Product1 : Product  Inputs=3
  Product2 : Product  Inputs=3
  Scope1 : Scope  NumInputPorts=3
  GearTrq [Nm] : Outport
  Gear [-] : Outport  Port=2
  wires:
  EngTrq [Nm]/1 -> Scope1/2, Product2/1
  Product1/1 -> Product2/2, Scope1/1, Gear [-]/1
  Product2/1 -> Scope1/3, GearTrq [Nm]/1
  Bus Selector/3 -> 1-D Lookup Table2/1  "<GearACmd>"
  GearCmd[-]/1 -> Bus Selector/1
  Bus Selector/1 -> 1-D Lookup Table3/1  "<FastSlowCmd>"
  Bus Selector/2 -> 1-D Lookup Table1/1  "<GearMCmd>"
  Effi/1 -> Product2/3
  1-D Lookup Table3/1 -> Product1/1
  1-D Lookup Table1/1 -> Product1/2
  1-D Lookup Table2/1 -> Product1/3

== system Tractor_HIT_Discrete/WorkloadModel/Transmission/GearBox2Axle ==
  note: 主减速比
  note: 前桥减速比
  DriveCmd [-] : Inport
  GearTrq [Nm] : Inport  Port=2
  Gear [-] : Inport  Port=3
  PTOTrq [Nm] : Inport  Port=4
  LiftTrq [Nm] : Inport  Port=5
  4WD : Subsystem  TreatAsAtomicUnit=on
  Constant : Constant  Value=GearFront
  Constant1 : Constant  Value=GearRef
  Constant2 : Constant  Value=GearFront
  Constant3 : Constant  Value=GearRef
  If : If  IfExpression=u1 == 0  ElseIfExpressions=u1 == 1  ShowElse=off
  Merge : Merge
  Merge1 : Merge
  Product{,1..3} (4 alike) : Product
  RWD : Subsystem  TreatAsAtomicUnit=on
  Scope1 : Scope  NumInputPorts=3
  Scope2 : Scope  NumInputPorts=4
  Subtract : Sum  Inputs=+--
  AxlTrqF [Nm] : Outport
  AxlTrqR [Nm] : Outport  Port=2
  Gear_F[-] : Outport  Port=3
  Gear_R[-] : Outport  Port=4
  wires:
  RWD/2(AxlTrqR [Nm]) -> Merge/1
  4WD/1(AxlTrqF [Nm]) -> Merge1/2
  DriveCmd [-]/1 -> If/1
  If/2 -> 4WD/Action
  PTOTrq [Nm]/1 -> Subtract/2
  RWD/1(AxlTrqF [Nm]) -> Merge1/1
  If/1 -> RWD/Action
  GearTrq [Nm]/1 -> Scope2/1, Subtract/1
  4WD/2(AxlTrqR [Nm]) -> Merge/2
  LiftTrq [Nm]/1 -> Subtract/3
  Subtract/1 -> Scope2/2, RWD/1(AxlTrq [Nm]), 4WD/1(AxlTrq [Nm])
  Gear [-]/1 -> Scope1/1, Product/1, Product1/1
  Product1/1 -> Scope1/2, Gear_F[-]/1
  Product/1 -> Scope1/3, Gear_R[-]/1
  Constant/1 -> Product1/2
  Constant1/1 -> Product/2
  Merge1/1 -> Product2/1
  Product2/1 -> Scope2/3, AxlTrqF [Nm]/1
  Constant2/1 -> Product2/2
  Constant3/1 -> Product3/2
  Merge/1 -> Product3/1
  Product3/1 -> Scope2/4, AxlTrqR [Nm]/1

== system Tractor_HIT_Discrete/WorkloadModel/Transmission/Motion ==
  EngineTrq_Nm : Inport
  LoadTrq_Nm : Inport  Port=2
  Add : Sum  Inputs=+-
  Constant : Constant  Value=Inertia
  Constant1 : Constant  Value=radps2rpm
  Divide : Product  Inputs=*/
  Integrator : Integrator  InitialCondition=SpeedInit  LimitOutput=on  UpperSaturationLimit=2400  LowerSaturationLimit=700
  Mux : Mux  Inputs=2
  Product : Product
  Scope2 : Scope  NumInputPorts=2
  EngineSpd_rpm : Outport
  wires:
  EngineTrq_Nm/1 -> Mux/1, Add/1
  LoadTrq_Nm/1 -> Mux/2, Add/2
  Add/1 -> Divide/1
  Constant/1 -> Divide/2
  Constant1/1 -> Product/2
  Product/1 -> Integrator/1
  Divide/1 -> Product/1
  Integrator/1 -> Scope2/2, EngineSpd_rpm/1
  Mux/1 -> Scope2/1

== system Tractor_HIT_Discrete/Engine/Engine/AftertreatmentModel/DOC ==
  note: GHSV = 气体空速，Gas Hourly Space Velocity
  ExhMassFlow_kg/h : Inport
  EGT_c : Inport  Port=2
  ExhPrs_kpa : Inport  Port=3
  O2_pct : Inport  Port=4
  NOx_kg/h : Inport  Port=5
  HC_kg/h : Inport  Port=6
  CO_kg/h : Inport  Port=7
  PM_kg/h : Inport  Port=8
  Add{,1..2,4} (4 alike) : Sum  Inputs=+-
  Add3 : Sum  Inputs=+++
  Constant : Constant
  Constant1 : Constant
  Constant2 : Constant
  DOCdPrs : Lookup_n-D  NumberOfTableDimensions=1  BreakpointsForDimension1=DOCdPrs_x  Table=DOCdPrs  ExtrapMethod=Clip  InternalRulePriority=Speed  RndMeth=Simplest
  GHSV : Subsystem
  Gain : Gain  Gain=20
  Gain1 : Gain  Gain=25
  Product{,1..3} (4 alike) : Product
  Scope : Scope  NumInputPorts=4
  Terminator : Terminator
  eta_CO : Lookup_n-D  BreakpointsForDimension1=etaCO_x  BreakpointsForDimension2=etaCO_y  Table=etaCO  ExtrapMethod=Clip  InternalRulePriority=Speed  RndMeth=Simplest
      settings: InputPortMap=u0,u1
  eta_HC : Lookup_n-D  BreakpointsForDimension1=etaHC_x  BreakpointsForDimension2=etaHC_y  Table=etaHC  ExtrapMethod=Clip  InternalRulePriority=Speed  RndMeth=Simplest
      settings: InputPortMap=u0,u1
  eta_NO2 : Lookup_n-D  BreakpointsForDimension1=etaNO2_x  BreakpointsForDimension2=etaNO2_y  Table=etaNO2  ExtrapMethod=Clip  InternalRulePriority=Speed  RndMeth=Simplest
      settings: InputPortMap=u0,u1
  DOC_Flow_kg/h : Outport
  DOC_Temp_c : Outport  Port=2
  DOC_NO2Frac : Outport  Port=3
  DOC_PM_kg/h : Outport  Port=4
  DOC_NO2_kg/h : Outport  Port=5
  DOC_NO_kg/h : Outport  Port=6
  DOC_Prs_kpa : Outport  Port=7
  DOC_dPrs_kpa : Outport  Port=8
  DOC_HC_kg/h : Outport  Port=9
  DOC_CO_kg/h : Outport  Port=10
  wires:
  PM_kg/h/1 -> DOC_PM_kg/h/1
  ExhPrs_kpa/1 -> DOCdPrs/1, Add4/1, GHSV/3(ExhPrs_kpa)
  EGT_c/1 -> Add3/3, eta_NO2/2, eta_HC/2, eta_CO/2, GHSV/2(EGT_c)
  ExhMassFlow_kg/h/1 -> GHSV/1(ExhMassFlow_kg/h), DOC_Flow_kg/h/1
  GHSV/1(GHSV_1/h) -> eta_NO2/1, eta_HC/1, eta_CO/1
  eta_CO/1 -> Gain/1, Add/2
  Constant/1 -> Add/1
  Add/1 -> Product/2
  CO_kg/h/1 -> Product/1
  Product/1 -> Scope/1, DOC_CO_kg/h/1  "DOC_CO_kg"
  Product1/1 -> Scope/2, DOC_HC_kg/h/1  "DOC_HC_kg/h"
  Add1/1 -> Product1/2
  Constant1/1 -> Add1/1
  eta_HC/1 -> Gain1/1, Add1/2
  HC_kg/h/1 -> Product1/1
  NOx_kg/h/1 -> Product3/1, Product2/2
  Product2/1 -> Scope/3, DOC_NO2_kg/h/1  "DOC_NO2_kg/h"
  Product3/1 -> Scope/4, DOC_NO_kg/h/1  "DOC_NO_kg/h"
  eta_NO2/1 -> DOC_NO2Frac/1, Product2/1, Add2/2
  Constant2/1 -> Add2/1
  Add2/1 -> Product3/2
  O2_pct/1 -> Terminator/1
  DOCdPrs/1 -> Add4/2, DOC_dPrs_kpa/1
  Gain/1 -> Add3/1
  Gain1/1 -> Add3/2
  Add3/1 -> DOC_Temp_c/1
  Add4/1 -> DOC_Prs_kpa/1

== system Tractor_HIT_Discrete/Engine/Engine/AftertreatmentModel/DPF ==
  DOC_Flow_kg/h : Inport
  DOC_Temp_c : Inport  Port=2
  DOC_NO2Frac : Inport  Port=3
  DOC_PM_kg/h : Inport  Port=4
  DOC_NO2_kg/h : Inport  Port=5
  DOC_NO_kg/h : Inport  Port=6
  DOC_Prs_kpa : Inport  Port=7
  DPF_regen_req : Inport  Port=8
  Add : Sum  Inputs=+-
  Add1 : Sum
  Add4 : Sum  Inputs=-+
  Constant : Constant
  DPFdPrs : Lookup_n-D  BreakpointsForDimension1=DPFdPrs_x  BreakpointsForDimension2=DPFdPrs_y  Table=DPFdPrs  InternalRulePriority=Speed  RndMeth=Simplest
      settings: InputPortMap=u0,u1
  GHSV : Subsystem
  Product : Product
  Scope : Scope  NumInputPorts=2
  SootLoad : Subsystem
  eta_PM : Lookup_n-D  BreakpointsForDimension1=etaPM_x  BreakpointsForDimension2=etaPM_y  Table=etaPM  InternalRulePriority=Speed  RndMeth=Simplest
      settings: InputPortMap=u0,u1
  DPF_Flow_kg/h : Outport
  DPF_Temp_c : Outport  Port=2
  DPF_Prs_kpa : Outport  Port=3
  DPF_NOx_kg/h : Outport  Port=4
  DPF_NO2Frac : Outport  Port=5
  DPF_PM_kg/h : Outport  Port=6
  DPF_SootLoad_g : Outport  Port=7
  DPF_dPrs_kpa : Outport  Port=8
  wires:
  DOC_NO2Frac/1 -> DPF_NO2Frac/1
  DOC_Flow_kg/h/1 -> DPFdPrs/1, DPF_Flow_kg/h/1, GHSV/1(ExhMassFlow_kg/h), SootLoad/2(DOC_Flow_kg/h)
  DOC_Temp_c/1 -> GHSV/2(EGT_c), SootLoad/3(DOC_Temp_c), DPF_Temp_c/1, eta_PM/2
  DOC_Prs_kpa/1 -> Add4/2, GHSV/3(ExhPrs_kpa)
  GHSV/1(GHSV_1/h) -> eta_PM/1
  Product/1 -> Scope/1, DPF_PM_kg/h/1
  Constant/1 -> Add/1
  eta_PM/1 -> SootLoad/4(eta_PM), Add/2
  Add/1 -> Product/1
  DOC_PM_kg/h/1 -> Scope/2, SootLoad/5(DOC_PM_kg/h), Product/2
  DPF_regen_req/1 -> SootLoad/1(DPF_regen_req)
  SootLoad/1(SootLoad_g) -> DPFdPrs/2, DPF_SootLoad_g/1
  DPFdPrs/1 -> Add4/1, DPF_dPrs_kpa/1
  Add4/1 -> DPF_Prs_kpa/1
  DOC_NO2_kg/h/1 -> Add1/1
  DOC_NO_kg/h/1 -> Add1/2
  Add1/1 -> DPF_NOx_kg/h/1

== system Tractor_HIT_Discrete/Engine/Engine/AftertreatmentModel/SCR ==
  note: 0.0001~0.001 kg/h 这个量级
  note: SCR 载体内部积存的氨，是积分状态；
  note: 氨逃逸
  note: 实际尿素喷射流量
  note: 尿素喷射执行
  DPF_Flow_kg/h : Inport
  DPF_Temp_c : Inport  Port=2
  DPF_Prs_kpa : Inport  Port=3
  DPF_NOx_kg/h : Inport  Port=4
  mUREA_target : Inport  Port=5
  Add1 : Sum  Inputs=+--
  Add2 : Sum  Inputs=+-
  Add3 : Sum  Inputs=+-
  Integrator : Integrator  UpperSaturationLimit=NH3_MAX  LowerSaturationLimit=0
  NH3StoreMax : Lookup_n-D  NumberOfTableDimensions=1  BreakpointsForDimension1=NH3StoreMax_x  Table=NH3StoreMax  ExtrapMethod=Clip  InternalRulePriority=Speed  RndMeth=Simplest
  Product1 : Product
  Product2 : Product
  Product3 : Product
  SCRdPrs : Lookup_n-D  BreakpointsForDimension1=SCRdPrs_x  BreakpointsForDimension2=SCRdPrs_y  Table=SCRdPrs  ExtrapMethod=Clip  InternalRulePriority=Speed  RndMeth=Simplest
      settings: InputPortMap=u0,u1
  Saturation Dynamic1 : simulink/Discontinuities/Saturation Dynamic  OutMin=[]  OutMax=[]  OutDataTypeStr=Inherit: Same as second input  OutDataType=fixdt(1, 16)  OutScaling=2^-10  DoSatur=off
  Scope : Scope  NumInputPorts=6
  Transfer Fcn : TransferFcn  Denominator=[1 1]
  eta_NOx : Lookup_n-D  BreakpointsForDimension1=etaPM_x  BreakpointsForDimension2=etaPM_y  Table=etaPM  ExtrapMethod=Clip  InternalRulePriority=Speed  RndMeth=Simplest
      settings: InputPortMap=u0,u1
  kg/h2g/s : Gain  Gain=1000/3600
  one : Constant
  zero3 : Constant  Value=0
  zero4 : Constant  Value=0.0002
  尿素浓度1 : Constant  Value=0.325
  OUT_Flow_kg/h : Outport
  OUT_Temp_c : Outport  Port=2
  OUT_Prs_kpa : Outport  Port=3
  OUT_NOx_kg/h : Outport  Port=4
  OUT_mNH3_slip : Outport  Port=5
  OUT_NH3store_g : Outport  Port=6
  wires:
  DPF_NOx_kg/h/1 -> Scope/1, Product2/1, Product3/2  "DPF_NOx_kg/hm_NOx"
  DPF_Flow_kg/h/1 -> eta_NOx/1, [DPF_Flow], OUT_Flow_kg/h/1
  DPF_Temp_c/1 -> eta_NOx/2, OUT_Temp_c/1, [DPF_Temp_c]
  eta_NOx/1 -> Add2/2, Product2/2  "etaNOx"
  Transfer Fcn/1 -> Product1/1  "mUREA"
  Product1/1 -> Add1/1, Scope/3  "mNH3_in"
  Product2/1 -> Add1/2  "mNH3_consume"
  kg/h2g/s/1 -> Scope/5, Integrator/1  "OUT_NH3storeRate_g/s"
  Saturation Dynamic1/1 -> Scope/6, OUT_NH3store_g/1, SCRdPrs/2  "NH3_store"
  SCRdPrs/1 -> Add3/2  "SCR_dPrs"
  DPF_Prs_kpa/1 -> Add3/1
  Add3/1 -> OUT_Prs_kpa/1
  Integrator/1 -> Saturation Dynamic1/2
  zero3/1 -> Saturation Dynamic1/3
  [DPF_Temp_c] -> NH3StoreMax/1
  NH3StoreMax/1 -> Saturation Dynamic1/1
  [DPF_Flow] -> SCRdPrs/1
  zero4/1 -> Scope/4, OUT_mNH3_slip/1, Add1/3  "mNH3_slip"
  one/1 -> Add2/1
  Add2/1 -> Product3/1
  Product3/1 -> Scope/2, OUT_NOx_kg/h/1  "OUT_NOx_kg/h"
  尿素浓度1/1 -> Product1/2
  mUREA_target/1 -> Transfer Fcn/1
  Add1/1 -> kg/h2g/s/1
